simulink model "sf_edgetrigger_approx_fcncall"  (R2025b)
settings: Solver=FixedStepDiscrete  StartTime=0.0  StopTime=40  FixedStep=1.0  RelTol=1e-3  EnableMultiTasking=on
settings Model: Creator=The MathWorks, Inc.  LastModifiedBy=The MathWorks, Inc.
settings SolverCC: AlgebraicLoopSolver=TrustRegion
settings DataIOCC: LimitDataPoints=on  SaveFormat=Array  ReturnWorkspaceOutputs=off
settings OptimizationCC: ReuseModelBlockBuffer=off  ExpressionDepthLimit=2147483647.0  LifeSpan=inf
settings DebuggingCC: UnderspecifiedInitializationDetection=Classic  MergeDetectMultiDrivingBlocksExec=none  SolverPrmCheckMsg=warning  FcnCallInpInsideContextMsg=warning  UnconnectedInputMsg=warning  UnconnectedOutputMsg=warning  UnconnectedLineMsg=warning  StateNameClashWarn=warning  SFUnexpectedBacktrackingDiag=warning  SFNoUnconditionalDefaultTransitionDiag=warning  SFExecutionAtInitializationDiag=none  ArithmeticOperatorsInVariantConditions=warning
settings HardwareCC: ProdBitPerPointer=32.0  ProdBitPerSizeT=32.0  ProdBitPerPtrDiffT=32.0  ProdLargestAtomicFloat=None  ProdIntDivRoundTo=Undefined  ProdEndianess=Unspecified  ProdWordSize=32.0  ProdHWDeviceType=32-bit Generic
settings ModelReferenceCC: EnableRefExpFcnMdlSchedulingChecks=on  PropagateSignalLabelsOutOfModel=off
settings SFSimCC: SimUseLocalCustomCode=off  SimParseCustomCode=off  CustomCodeUndefinedFunction=UseInterfaceOnly
settings RTWCC: RTWUseLocalCustomCode=off  GPUComputeCapability=3.5
settings CodeAppCC: StateflowObjectComments=on
settings GRTTargetCC: TargetLangStandard=C89/C90 (ANSI)  CombineOutputUpdateFcns=off  GRTInterface=on
settings ConfigComp: CovMetricSettings=dw  CovSaveCumulativeToWorkspaceVar=on  CovSaveSingleToWorkspaceVar=on  CovExternalEMLEnable=off

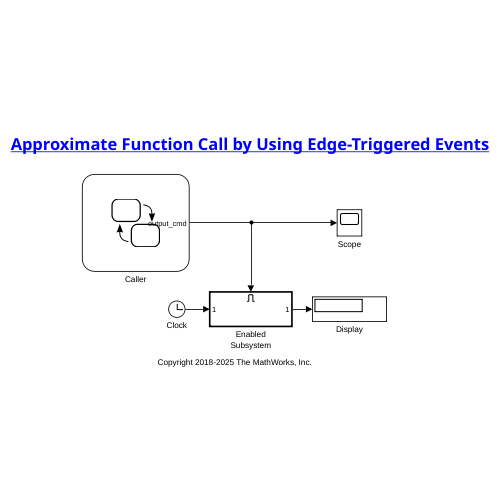
[thumbnail: Simulink's stored preview of the top-level diagram]
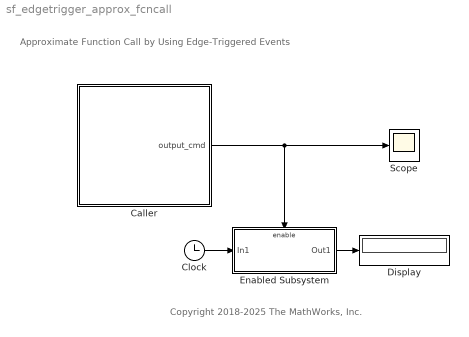
== system sf_edgetrigger_approx_fcncall ==
  note: Copyright 2018-2025 The MathWorks, Inc.
  note: Approximate Function Call by Using Edge-Triggered Events
  Caller : Stateflow chart  TreatAsAtomicUnit=on
  Clock : Clock
  Display : Display
  Enabled Subsystem : Subsystem  TreatAsAtomicUnit=on
  Scope : Scope
      settings: TimeSpan=40  ActiveDisplayYMinimum=-1  ActiveDisplayYMaximum=2
  wires:
  Caller/1(output_cmd) -> Enabled Subsystem/Enable, Scope/1
  Clock/1 -> Enabled Subsystem/1(In1)
  Enabled Subsystem/1(Out1) -> Display/1

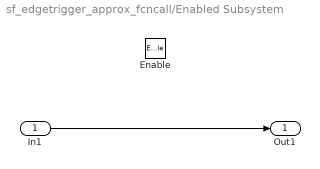
== system sf_edgetrigger_approx_fcncall/Enabled Subsystem ==
  In1 : Inport
  Enable : EnablePort
  Out1 : Outport  VectorParamsAs1DForOutWhenUnconnected=off
  wires:
  In1/1 -> Out1/1

== stateflow chart sf_edgetrigger_approx_fcncall/Caller ==
  state Start
  state End
  (default) -> Start
  Start -> End : [after(20,sec)] {send(output_cmd)}
  events: output_cmd output EITHER_EDGE_EVENT
